simulink model "ss1_power_plant"  (R2024b)
settings: Solver=ode45  StartTime=0.0  StopTime=0.1  MaxStep=1  MinStep=0.001  RelTol=1e-3
undefined symbols (not defined in the file): BAT, PV
settings Model: Creator=user  LastModifiedBy=user

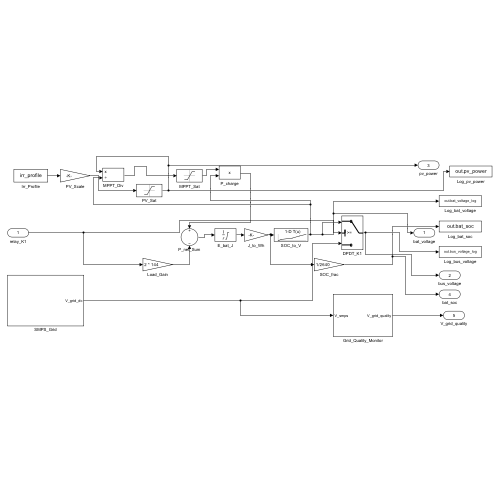
[thumbnail: Simulink's stored preview of the top-level diagram]
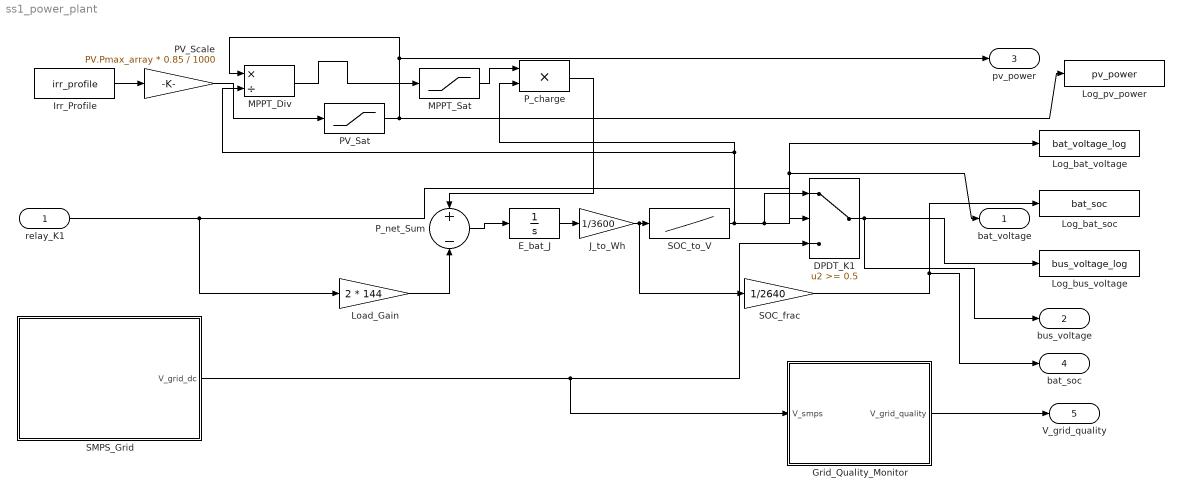
== system ss1_power_plant ==
  relay_K1 : Inport
  DPDT_K1 : Switch  Threshold=0.5  SaturateOnIntegerOverflow=off  InputSameDT=off
  E_bat_J : Integrator  InitialCondition=BAT.initial_soc * BAT.capacity_wh * 3600  LimitOutput=on  UpperSaturationLimit=BAT.capacity_wh * 3600  LowerSaturationLimit=0
  Grid_Quality_Monitor : Subsystem
  Irr_Profile : FromWorkspace  VariableName=irr_profile
  J_to_Wh : Gain  Gain=1/3600
  Load_Gain : Gain  Gain=2 * 144
  Log_bat_soc : ToWorkspace  VariableName=bat_soc  SampleTime=-1
  Log_bat_voltage : ToWorkspace  VariableName=bat_voltage_log  SampleTime=-1
  Log_bus_voltage : ToWorkspace  VariableName=bus_voltage_log  SampleTime=-1
  Log_pv_power : ToWorkspace  VariableName=pv_power  SampleTime=-1
  MPPT_Div : Product  Inputs=*/
  MPPT_Sat : Saturate  UpperLimit=150  LowerLimit=0
  PV_Sat : Saturate  UpperLimit=PV.Pmax_array  LowerLimit=0
  PV_Scale : Gain  Gain=PV.Pmax_array * 0.85 / 1000
  P_charge : Product
  P_net_Sum : Sum  Inputs=+-
  SMPS_Grid : Subsystem
  SOC_frac : Gain  Gain=1/2640
  SOC_to_V : Lookup_n-D  NumberOfTableDimensions=1  BreakpointsForDimension1=[0, 264, 1320, 1980, 2640]  Table=[11.6, 11.8, 12.0, 12.4, 12.7]  ExtrapMethod=Clip  InternalRulePriority=Speed  RndMeth=Simplest
  bat_voltage : Outport
  bus_voltage : Outport  Port=2
  pv_power : Outport  Port=3
  bat_soc : Outport  Port=4
  V_grid_quality : Outport  Port=5
  wires:
  Irr_Profile/1 -> PV_Scale/1
  PV_Scale/1 -> PV_Sat/1
  PV_Sat/1 -> Log_pv_power/1, MPPT_Div/1, pv_power/1
  SOC_to_V/1 -> Log_bat_voltage/1, bat_voltage/1, DPDT_K1/1, MPPT_Div/2, P_charge/2
  MPPT_Div/1 -> MPPT_Sat/1
  MPPT_Sat/1 -> P_charge/1
  P_charge/1 -> P_net_Sum/1
  relay_K1/1 -> Load_Gain/1, DPDT_K1/2
  Load_Gain/1 -> P_net_Sum/2
  P_net_Sum/1 -> E_bat_J/1
  E_bat_J/1 -> J_to_Wh/1
  J_to_Wh/1 -> SOC_to_V/1, SOC_frac/1
  DPDT_K1/1 -> bus_voltage/1, Log_bus_voltage/1
  SOC_frac/1 -> bat_soc/1, Log_bat_soc/1
  SMPS_Grid/1(V_grid_dc) -> Grid_Quality_Monitor/1(V_smps), DPDT_K1/3
  Grid_Quality_Monitor/1(V_grid_quality) -> V_grid_quality/1

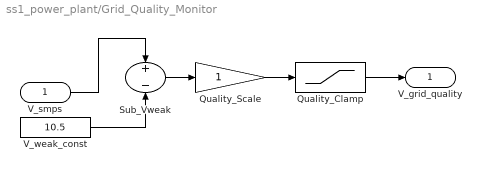
== system ss1_power_plant/Grid_Quality_Monitor ==
  V_smps : Inport
  Quality_Clamp : Saturate  UpperLimit=1  LowerLimit=0
  Quality_Scale : Gain
  Sub_Vweak : Sum  Inputs=+-
  V_weak_const : Constant  Value=10.5
  V_grid_quality : Outport
  wires:
  V_smps/1 -> Sub_Vweak/1
  V_weak_const/1 -> Sub_Vweak/2
  Sub_Vweak/1 -> Quality_Scale/1
  Quality_Scale/1 -> Quality_Clamp/1
  Quality_Clamp/1 -> V_grid_quality/1

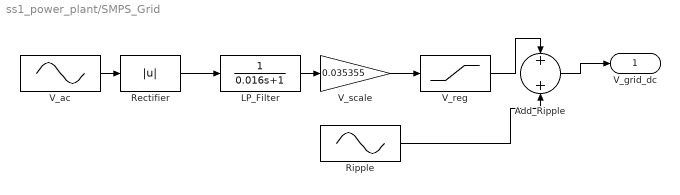
== system ss1_power_plant/SMPS_Grid ==
  Add_Ripple : Sum
  LP_Filter : TransferFcn  Denominator=[0.016 1]
  Rectifier : Abs  SaturateOnIntegerOverflow=off
  Ripple : Sin  Amplitude=0.12  Frequency=628.3185  SampleTime=0
  V_ac : Sin  Amplitude=339.4112549695428  Frequency=0  SampleTime=0
  V_reg : Saturate  UpperLimit=12  LowerLimit=0
  V_scale : Gain  Gain=0.035355
  V_grid_dc : Outport
  wires:
  V_ac/1 -> Rectifier/1
  Rectifier/1 -> LP_Filter/1
  LP_Filter/1 -> V_scale/1
  V_scale/1 -> V_reg/1
  V_reg/1 -> Add_Ripple/1
  Ripple/1 -> Add_Ripple/2
  Add_Ripple/1 -> V_grid_dc/1
